simulink model "electronic_speed_controller"  (R2024b)
settings: Solver=VariableStepAuto  StartTime=0.0  StopTime=10.0  RelTol=1e-3
undefined symbols (not defined in the file): plecs
libraries: autolibbldc x1
settings Model: Creator=jarre  LastModifiedBy=jarre

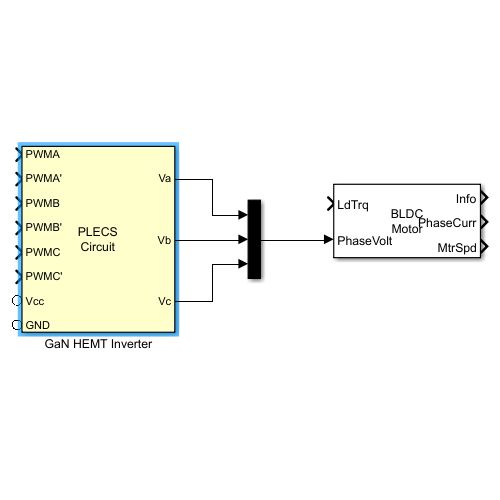
[thumbnail: Simulink's stored preview of the top-level diagram]
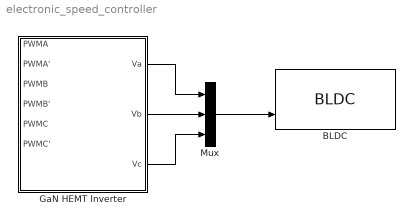
== system electronic_speed_controller ==
  BLDC : autolibbldc/BLDC  VariantControl=pmsmVariant==pmsmEnum.TorqueInput  MechInput=Torque  SimType=Continuous  BlockSampleTime=25e-6  p=4  Rs=0.36  Ld=2e-4  Lq=2e-4  Lambda=0.0064  J=7.0616e-06  B=2.6369e-06  F=0  Id_init=0  Iq_init=0  Th_init=0  Omega_init=0  RefBlkName='autolibbldc/BLDC'  aMode=5
      settings: LibrarySourceBlock=mcblib/Electrical Systems/Motors/BLDC
  GaN HEMT Inverter : Subsystem  LoadFcn=plecs('sl', 200);  InitFcn=plecs('sl', 214);  StartFcn=plecs('sl', 208);  StopFcn=plecs('sl', 209);  mask(PlecsCircuit){PLECSData=<binary blob, 2432 chars, not shown>}
      mask prompts: PLECSData "PLECS Data (Do not delete or modify!)"
      mask init:
      | % PLACE CUSTOM INITIALIZATIONS ABOVE
      | % DO NOT REMOVE
      | plecs('sl', 215);
      | % DO NOT REMOVE
      settings: CopyFcn=plecs('sl', 203);  DeleteFcn=plecs('sl', 205);  UndoDeleteFcn=plecs('sl', 206);  PreSaveFcn=plecs('sl', 211);  PostSaveFcn=plecs('sl', 201);  NameChangeFcn=plecs('sl', 210);  DestroyFcn=plecs('sl', 207);  PreCopyFcn=plecs('sl', 216);  OpenFcn=plecs('sl', 202);  ErrorFcn=plerrorfcn
      mask Help: eval('plecs(''help'', ''qthelp:///creatingacircuit.html'')')
      mask Display: disp('PLECS\nCircuit')
  Mux : Mux  Inputs=3
  wires:
  GaN HEMT Inverter/1(Va) -> Mux/1
  GaN HEMT Inverter/2(Vb) -> Mux/2
  GaN HEMT Inverter/3(Vc) -> Mux/3
  Mux/1 -> BLDC/2

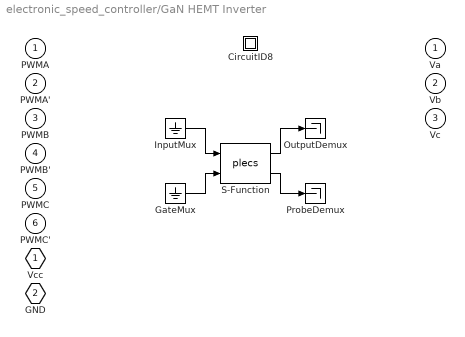
== system electronic_speed_controller/GaN HEMT Inverter ==
  PWMA : Inport
  PWMA' : Inport  Port=2
  PWMB : Inport  Port=3
  PWMB' : Inport  Port=4
  PWMC : Inport  Port=5
  PWMC' : Inport  Port=6
  " CircuitID8 " : Subsystem
  " GateMux " : Ground
  " InputMux " : Ground
  " OutputDemux " : Terminator
  " ProbeDemux " : Terminator
  " S-Function " : S-Function  FunctionName=plecs  SFunctionDeploymentMode=off  EnableBusSupport=off
  Vcc : PMIOPort  Side=Left
  GND : PMIOPort  Port=2  Side=Left
  Va : Outport
  Vb : Outport  Port=2
  Vc : Outport  Port=3
  wires:
  " S-Function "/1 -> " OutputDemux "/1
  " InputMux "/1 -> " S-Function "/1
  " GateMux "/1 -> " S-Function "/2
  " S-Function "/2 -> " ProbeDemux "/1

== system electronic_speed_controller/GaN HEMT Inverter/ CircuitID8  ==
